simulink model "s_c_nbe_m1k"  (R2016b)
settings: Solver=VariableStepAuto  StartTime=0.0  StopTime=1000  RelTol=1e-3  EnableMultiTasking=on
undefined symbols (not defined in the file): Coeffs, fft_stages, n_taps, output_bits, pfb_coeff_gen_calc, xengbits
libraries: xbsIndex_r4 x23639, casper_library_misc x65, casper_library_scopes x4, xbsReplacements_r4 x4, xps_library x3
(part 34 of 198)

== system s_c_nbe_m1k/DDC/dec_fir_async1 ==
  sync_in : Inport
  dv_in : Inport  Port=2
  real1 : Inport  Port=3
  imag1 : Inport  Port=4
  real2 : Inport  Port=5
  imag2 : Inport  Port=6
  real3 : Inport  Port=7
  imag3 : Inport  Port=8
  real4 : Inport  Port=9
  imag4 : Inport  Port=10
  real5 : Inport  Port=11
  imag5 : Inport  Port=12
  real6 : Inport  Port=13
  imag6 : Inport  Port=14
  real7 : Inport  Port=15
  imag7 : Inport  Port=16
  real8 : Inport  Port=17
  imag8 : Inport  Port=18
  convert1 : xbsIndex_r4/Convert  gui_display_data_type=Fixed-point  arith_type="Signed  (2's comp)"  n_bits=10  bin_pt=9  float_type=Single  exp_bits=8  fraction_bits=24  quantization="Round  (unbiased: +/- Inf)"  overflow=Wrap  en=off  latency=7  pipeline=off  dbl_ovrd=off  block_type=convert
  convert2 : xbsIndex_r4/Convert  gui_display_data_type=Fixed-point  arith_type="Signed  (2's comp)"  n_bits=10  bin_pt=9  float_type=Single  exp_bits=8  fraction_bits=24  quantization="Round  (unbiased: +/- Inf)"  overflow=Wrap  en=off  latency=7  pipeline=off  dbl_ovrd=off  block_type=convert
  dv_delay : xbsIndex_r4/Delay  rst=off  infoeditControl=Selection of Reset will increase slice count due to use of real FFs and instead of SRLs  en=off  latency=70  reg_retiming=off  dbl_ovrd=off  block_type=delay
      settings: infoedit=Hardware notes: A delay line is a chain, each link of which is an SRL16 or SRL32 followed by a flip-flop.
  fir_col_async1 : Subsystem  AncestorBlock=casper_library_downconverter/fir_col_async  mask(fir_col_async){n_inputs=8, coeff=[-0.00042458 -0.00037722 -0.00032902 -0.00028149 -0.00023577 -0.00019291 -0.00015346   -0.000271], add_latency=7, mult_latency=7, coeff_bit_width=18, coeff_bin_pt=17, first_stage_hdl=on, adder_imp=DSP48, async=on, bus_input=off, input_width=0, input_bp=0, input_type=Signed, dbl=on}
      mask prompts: n_inputs "Inputs"; coeff "Coefficients"; add_latency "Add latency"; mult_latency "Mult Latency"; coeff_bit_width "Coefficient bit width"; coeff_bin_pt "Coefficient binary point"; first_stage_hdl "Implement first stage of adder trees on output as behavioural HDL"; adder_imp "Adder implementation"; async "Asynchronous ops"; bus_input "Bus input"; input_width "Input bitwidth"; input_bp "Input binary point"; input_type "Input datatype"; dbl "Double col"
      mask init:
      | fir_col_async_init(gcb);
      mask Help: eval('xlWeb(''http://casper.berkeley.edu/wiki/Fir_col'')')
      mask TypeOptions adder_imp: Behavioral | Fabric | DSP48
      mask Callback bus_input:
      | onoff = get_param(gcb, 'bus_input');
      | set_param_state(gcb, 'input_width', onoff)
      | set_param_state(gcb, 'input_bp', onoff)
      | set_param_state(gcb, 'input_type', onoff)
      mask TypeOptions input_type: Signed | Unsigned
  fir_col_async10 : Subsystem  AncestorBlock=casper_library_downconverter/fir_col_async  mask(fir_col_async){n_inputs=8, coeff=[0.0053089   0.0052932   0.0051518   0.0048953   0.0045363   0.0040891   0.0035695   0.0029938], add_latency=7, mult_latency=7, coeff_bit_width=18, coeff_bin_pt=17, first_stage_hdl=on, adder_imp=DSP48, async=on, bus_input=off, input_width=0, input_bp=0, input_type=Signed, dbl=on}
      mask prompts: n_inputs "Inputs"; coeff "Coefficients"; add_latency "Add latency"; mult_latency "Mult Latency"; coeff_bit_width "Coefficient bit width"; coeff_bin_pt "Coefficient binary point"; first_stage_hdl "Implement first stage of adder trees on output as behavioural HDL"; adder_imp "Adder implementation"; async "Asynchronous ops"; bus_input "Bus input"; input_width "Input bitwidth"; input_bp "Input binary point"; input_type "Input datatype"; dbl "Double col"
      mask init:
      | fir_col_async_init(gcb);
      mask Help: eval('xlWeb(''http://casper.berkeley.edu/wiki/Fir_col'')')
      mask TypeOptions adder_imp: Behavioral | Fabric | DSP48
      mask Callback bus_input:
      | onoff = get_param(gcb, 'bus_input');
      | set_param_state(gcb, 'input_width', onoff)
      | set_param_state(gcb, 'input_bp', onoff)
      | set_param_state(gcb, 'input_type', onoff)
      mask TypeOptions input_type: Signed | Unsigned
  fir_col_async11 : Subsystem  AncestorBlock=casper_library_downconverter/fir_col_async  mask(fir_col_async){n_inputs=8, coeff=[0.00060481   0.0016168   0.0025297    0.003328   0.0039999   0.0045369   0.0049344   0.0051911], add_latency=7, mult_latency=7, coeff_bit_width=18, coeff_bin_pt=17, first_stage_hdl=on, adder_imp=DSP48, async=on, bus_input=off, input_width=0, input_bp=0, input_type=Signed, dbl=on}
      mask prompts: n_inputs "Inputs"; coeff "Coefficients"; add_latency "Add latency"; mult_latency "Mult Latency"; coeff_bit_width "Coefficient bit width"; coeff_bin_pt "Coefficient binary point"; first_stage_hdl "Implement first stage of adder trees on output as behavioural HDL"; adder_imp "Adder implementation"; async "Asynchronous ops"; bus_input "Bus input"; input_width "Input bitwidth"; input_bp "Input binary point"; input_type "Input datatype"; dbl "Double col"
      mask init:
      | fir_col_async_init(gcb);
      mask Help: eval('xlWeb(''http://casper.berkeley.edu/wiki/Fir_col'')')
      mask TypeOptions adder_imp: Behavioral | Fabric | DSP48
      mask Callback bus_input:
      | onoff = get_param(gcb, 'bus_input');
      | set_param_state(gcb, 'input_width', onoff)
      | set_param_state(gcb, 'input_bp', onoff)
      | set_param_state(gcb, 'input_type', onoff)
      mask TypeOptions input_type: Signed | Unsigned
  fir_col_async12 : Subsystem  AncestorBlock=casper_library_downconverter/fir_col_async  mask(fir_col_async){n_inputs=8, coeff=[-0.0082442  -0.0073287  -0.0062974  -0.0051819  -0.0040135  -0.0028225  -0.0016382 -0.00048749], add_latency=7, mult_latency=7, coeff_bit_width=18, coeff_bin_pt=17, first_stage_hdl=on, adder_imp=DSP48, async=on, bus_input=off, input_width=0, input_bp=0, input_type=Signed, dbl=on}
      mask prompts: n_inputs "Inputs"; coeff "Coefficients"; add_latency "Add latency"; mult_latency "Mult Latency"; coeff_bit_width "Coefficient bit width"; coeff_bin_pt "Coefficient binary point"; first_stage_hdl "Implement first stage of adder trees on output as behavioural HDL"; adder_imp "Adder implementation"; async "Asynchronous ops"; bus_input "Bus input"; input_width "Input bitwidth"; input_bp "Input binary point"; input_type "Input datatype"; dbl "Double col"
      mask init:
      | fir_col_async_init(gcb);
      mask Help: eval('xlWeb(''http://casper.berkeley.edu/wiki/Fir_col'')')
      mask TypeOptions adder_imp: Behavioral | Fabric | DSP48
      mask Callback bus_input:
      | onoff = get_param(gcb, 'bus_input');
      | set_param_state(gcb, 'input_width', onoff)
      | set_param_state(gcb, 'input_bp', onoff)
      | set_param_state(gcb, 'input_type', onoff)
      mask TypeOptions input_type: Signed | Unsigned
  fir_col_async13 : Subsystem  AncestorBlock=casper_library_downconverter/fir_col_async  mask(fir_col_async){n_inputs=8, coeff=[-0.0080689  -0.0090238   -0.009681   -0.010051   -0.010148  -0.0099918  -0.0096048  -0.0090129], add_latency=7, mult_latency=7, coeff_bit_width=18, coeff_bin_pt=17, first_stage_hdl=on, adder_imp=DSP48, async=on, bus_input=off, input_width=0, input_bp=0, input_type=Signed, dbl=on}
      mask prompts: n_inputs "Inputs"; coeff "Coefficients"; add_latency "Add latency"; mult_latency "Mult Latency"; coeff_bit_width "Coefficient bit width"; coeff_bin_pt "Coefficient binary point"; first_stage_hdl "Implement first stage of adder trees on output as behavioural HDL"; adder_imp "Adder implementation"; async "Asynchronous ops"; bus_input "Bus input"; input_width "Input bitwidth"; input_bp "Input binary point"; input_type "Input datatype"; dbl "Double col"
      mask init:
      | fir_col_async_init(gcb);
      mask Help: eval('xlWeb(''http://casper.berkeley.edu/wiki/Fir_col'')')
      mask TypeOptions adder_imp: Behavioral | Fabric | DSP48
      mask Callback bus_input:
      | onoff = get_param(gcb, 'bus_input');
      | set_param_state(gcb, 'input_width', onoff)
      | set_param_state(gcb, 'input_bp', onoff)
      | set_param_state(gcb, 'input_type', onoff)
      mask TypeOptions input_type: Signed | Unsigned
  fir_col_async14 : Subsystem  AncestorBlock=casper_library_downconverter/fir_col_async  mask(fir_col_async){n_inputs=8, coeff=[0.0097893   0.0067161    0.003832   0.0011688  -0.0012463  -0.0033914  -0.0052499  -0.0068109], add_latency=7, mult_latency=7, coeff_bit_width=18, coeff_bin_pt=17, first_stage_hdl=on, adder_imp=DSP48, async=on, bus_input=off, input_width=0, input_bp=0, input_type=Signed, dbl=on}
      mask prompts: n_inputs "Inputs"; coeff "Coefficients"; add_latency "Add latency"; mult_latency "Mult Latency"; coeff_bit_width "Coefficient bit width"; coeff_bin_pt "Coefficient binary point"; first_stage_hdl "Implement first stage of adder trees on output as behavioural HDL"; adder_imp "Adder implementation"; async "Asynchronous ops"; bus_input "Bus input"; input_width "Input bitwidth"; input_bp "Input binary point"; input_type "Input datatype"; dbl "Double col"
      mask init:
      | fir_col_async_init(gcb);
      mask Help: eval('xlWeb(''http://casper.berkeley.edu/wiki/Fir_col'')')
      mask TypeOptions adder_imp: Behavioral | Fabric | DSP48
      mask Callback bus_input:
      | onoff = get_param(gcb, 'bus_input');
      | set_param_state(gcb, 'input_width', onoff)
      | set_param_state(gcb, 'input_bp', onoff)
      | set_param_state(gcb, 'input_type', onoff)
      mask TypeOptions input_type: Signed | Unsigned
  fir_col_async15 : Subsystem  AncestorBlock=casper_library_downconverter/fir_col_async  mask(fir_col_async){n_inputs=8, coeff=[0.03623    0.033172    0.029949    0.026609    0.023197    0.019764    0.016355    0.013015], add_latency=7, mult_latency=7, coeff_bit_width=18, coeff_bin_pt=17, first_stage_hdl=on, adder_imp=DSP48, async=on, bus_input=off, input_width=0, input_bp=0, input_type=Signed, dbl=on}
      mask prompts: n_inputs "Inputs"; coeff "Coefficients"; add_latency "Add latency"; mult_latency "Mult Latency"; coeff_bit_width "Coefficient bit width"; coeff_bin_pt "Coefficient binary point"; first_stage_hdl "Implement first stage of adder trees on output as behavioural HDL"; adder_imp "Adder implementation"; async "Asynchronous ops"; bus_input "Bus input"; input_width "Input bitwidth"; input_bp "Input binary point"; input_type "Input datatype"; dbl "Double col"
      mask init:
      | fir_col_async_init(gcb);
      mask Help: eval('xlWeb(''http://casper.berkeley.edu/wiki/Fir_col'')')
      mask TypeOptions adder_imp: Behavioral | Fabric | DSP48
      mask Callback bus_input:
      | onoff = get_param(gcb, 'bus_input');
      | set_param_state(gcb, 'input_width', onoff)
      | set_param_state(gcb, 'input_bp', onoff)
      | set_param_state(gcb, 'input_type', onoff)
      mask TypeOptions input_type: Signed | Unsigned
  fir_col_async16 : Subsystem  AncestorBlock=casper_library_downconverter/fir_col_async  mask(fir_col_async){n_inputs=8, coeff=[0.050061     0.04964    0.048805    0.047569     0.04595    0.043974    0.041672    0.039077], add_latency=7, mult_latency=7, coeff_bit_width=18, coeff_bin_pt=17, first_stage_hdl=on, adder_imp=DSP48, async=on, bus_input=off, input_width=0, input_bp=0, input_type=Signed, dbl=on}
      mask prompts: n_inputs "Inputs"; coeff "Coefficients"; add_latency "Add latency"; mult_latency "Mult Latency"; coeff_bit_width "Coefficient bit width"; coeff_bin_pt "Coefficient binary point"; first_stage_hdl "Implement first stage of adder trees on output as behavioural HDL"; adder_imp "Adder implementation"; async "Asynchronous ops"; bus_input "Bus input"; input_width "Input bitwidth"; input_bp "Input binary point"; input_type "Input datatype"; dbl "Double col"
      mask init:
      | fir_col_async_init(gcb);
      mask Help: eval('xlWeb(''http://casper.berkeley.edu/wiki/Fir_col'')')
      mask TypeOptions adder_imp: Behavioral | Fabric | DSP48
      mask Callback bus_input:
      | onoff = get_param(gcb, 'bus_input');
      | set_param_state(gcb, 'input_width', onoff)
      | set_param_state(gcb, 'input_bp', onoff)
      | set_param_state(gcb, 'input_type', onoff)
      mask TypeOptions input_type: Signed | Unsigned
  fir_col_async2 : Subsystem  AncestorBlock=casper_library_downconverter/fir_col_async  mask(fir_col_async){n_inputs=8, coeff=[-0.00057574 -0.00059619   -0.000602 -0.00059433 -0.00057544  -0.0005472 -0.00051125 -0.00046978], add_latency=7, mult_latency=7, coeff_bit_width=18, coeff_bin_pt=17, first_stage_hdl=on, adder_imp=DSP48, async=on, bus_input=off, input_width=0, input_bp=0, input_type=Signed, dbl=on}
      mask prompts: n_inputs "Inputs"; coeff "Coefficients"; add_latency "Add latency"; mult_latency "Mult Latency"; coeff_bit_width "Coefficient bit width"; coeff_bin_pt "Coefficient binary point"; first_stage_hdl "Implement first stage of adder trees on output as behavioural HDL"; adder_imp "Adder implementation"; async "Asynchronous ops"; bus_input "Bus input"; input_width "Input bitwidth"; input_bp "Input binary point"; input_type "Input datatype"; dbl "Double col"
      mask init:
      | fir_col_async_init(gcb);
      mask Help: eval('xlWeb(''http://casper.berkeley.edu/wiki/Fir_col'')')
      mask TypeOptions adder_imp: Behavioral | Fabric | DSP48
      mask Callback bus_input:
      | onoff = get_param(gcb, 'bus_input');
      | set_param_state(gcb, 'input_width', onoff)
      | set_param_state(gcb, 'input_bp', onoff)
      | set_param_state(gcb, 'input_type', onoff)
      mask TypeOptions input_type: Signed | Unsigned
  fir_col_async3 : Subsystem  AncestorBlock=casper_library_downconverter/fir_col_async  mask(fir_col_async){n_inputs=8, coeff=[0.00024451  7.6958e-05 -7.3315e-05 -0.00020513 -0.00031757 -0.00041046 -0.00048394 -0.00053871], add_latency=7, mult_latency=7, coeff_bit_width=18, coeff_bin_pt=17, first_stage_hdl=on, adder_imp=DSP48, async=on, bus_input=off, input_width=0, input_bp=0, input_type=Signed, dbl=on}
      mask prompts: n_inputs "Inputs"; coeff "Coefficients"; add_latency "Add latency"; mult_latency "Mult Latency"; coeff_bit_width "Coefficient bit width"; coeff_bin_pt "Coefficient binary point"; first_stage_hdl "Implement first stage of adder trees on output as behavioural HDL"; adder_imp "Adder implementation"; async "Asynchronous ops"; bus_input "Bus input"; input_width "Input bitwidth"; input_bp "Input binary point"; input_type "Input datatype"; dbl "Double col"
      mask init:
      | fir_col_async_init(gcb);
      mask Help: eval('xlWeb(''http://casper.berkeley.edu/wiki/Fir_col'')')
      mask TypeOptions adder_imp: Behavioral | Fabric | DSP48
      mask Callback bus_input:
      | onoff = get_param(gcb, 'bus_input');
      | set_param_state(gcb, 'input_width', onoff)
      | set_param_state(gcb, 'input_bp', onoff)
      | set_param_state(gcb, 'input_type', onoff)
      mask TypeOptions input_type: Signed | Unsigned
  fir_col_async4 : Subsystem  AncestorBlock=casper_library_downconverter/fir_col_async  mask(fir_col_async){n_inputs=8, coeff=[0.0018729    0.001677     0.00147   0.0012565   0.0010415  0.00082907  0.00062325   0.0004274], add_latency=7, mult_latency=7, coeff_bit_width=18, coeff_bin_pt=17, first_stage_hdl=on, adder_imp=DSP48, async=on, bus_input=off, input_width=0, input_bp=0, input_type=Signed, dbl=on}
      mask prompts: n_inputs "Inputs"; coeff "Coefficients"; add_latency "Add latency"; mult_latency "Mult Latency"; coeff_bit_width "Coefficient bit width"; coeff_bin_pt "Coefficient binary point"; first_stage_hdl "Implement first stage of adder trees on output as behavioural HDL"; adder_imp "Adder implementation"; async "Asynchronous ops"; bus_input "Bus input"; input_width "Input bitwidth"; input_bp "Input binary point"; input_type "Input datatype"; dbl "Double col"
      mask init:
      | fir_col_async_init(gcb);
      mask Help: eval('xlWeb(''http://casper.berkeley.edu/wiki/Fir_col'')')
      mask TypeOptions adder_imp: Behavioral | Fabric | DSP48
      mask Callback bus_input:
      | onoff = get_param(gcb, 'bus_input');
      | set_param_state(gcb, 'input_width', onoff)
      | set_param_state(gcb, 'input_bp', onoff)
      | set_param_state(gcb, 'input_type', onoff)
      mask TypeOptions input_type: Signed | Unsigned
  fir_col_async5 : Subsystem  AncestorBlock=casper_library_downconverter/fir_col_async  mask(fir_col_async){n_inputs=8, coeff=[0.002468   0.0025259   0.0025398   0.0025118   0.0024451   0.0023435   0.0022111   0.0020526], add_latency=7, mult_latency=7, coeff_bit_width=18, coeff_bin_pt=17, first_stage_hdl=on, adder_imp=DSP48, async=on, bus_input=off, input_width=0, input_bp=0, input_type=Signed, dbl=on}
      mask prompts: n_inputs "Inputs"; coeff "Coefficients"; add_latency "Add latency"; mult_latency "Mult Latency"; coeff_bit_width "Coefficient bit width"; coeff_bin_pt "Coefficient binary point"; first_stage_hdl "Implement first stage of adder trees on output as behavioural HDL"; adder_imp "Adder implementation"; async "Asynchronous ops"; bus_input "Bus input"; input_width "Input bitwidth"; input_bp "Input binary point"; input_type "Input datatype"; dbl "Double col"
      mask init:
      | fir_col_async_init(gcb);
      mask Help: eval('xlWeb(''http://casper.berkeley.edu/wiki/Fir_col'')')
      mask TypeOptions adder_imp: Behavioral | Fabric | DSP48
      mask Callback bus_input:
      | onoff = get_param(gcb, 'bus_input');
      | set_param_state(gcb, 'input_width', onoff)
      | set_param_state(gcb, 'input_bp', onoff)
      | set_param_state(gcb, 'input_type', onoff)
      mask TypeOptions input_type: Signed | Unsigned
  fir_col_async6 : Subsystem  AncestorBlock=casper_library_downconverter/fir_col_async  mask(fir_col_async){n_inputs=8, coeff=[0.00046831  0.00084053   0.0011876   0.0015031   0.0017821   0.0020204   0.0022151   0.0023645], add_latency=7, mult_latency=7, coeff_bit_width=18, coeff_bin_pt=17, first_stage_hdl=on, adder_imp=DSP48, async=on, bus_input=off, input_width=0, input_bp=0, input_type=Signed, dbl=on}
      mask prompts: n_inputs "Inputs"; coeff "Coefficients"; add_latency "Add latency"; mult_latency "Mult Latency"; coeff_bit_width "Coefficient bit width"; coeff_bin_pt "Coefficient binary point"; first_stage_hdl "Implement first stage of adder trees on output as behavioural HDL"; adder_imp "Adder implementation"; async "Asynchronous ops"; bus_input "Bus input"; input_width "Input bitwidth"; input_bp "Input binary point"; input_type "Input datatype"; dbl "Double col"
      mask init:
      | fir_col_async_init(gcb);
      mask Help: eval('xlWeb(''http://casper.berkeley.edu/wiki/Fir_col'')')
      mask TypeOptions adder_imp: Behavioral | Fabric | DSP48
      mask Callback bus_input:
      | onoff = get_param(gcb, 'bus_input');
      | set_param_state(gcb, 'input_width', onoff)
      | set_param_state(gcb, 'input_bp', onoff)
      | set_param_state(gcb, 'input_type', onoff)
      mask TypeOptions input_type: Signed | Unsigned
  fir_col_async7 : Subsystem  AncestorBlock=casper_library_downconverter/fir_col_async  mask(fir_col_async){n_inputs=8, coeff=[-0.0024155   -0.002151  -0.0018401  -0.0014922  -0.0011167 -0.00072347  -0.0003221   7.805e-05], add_latency=7, mult_latency=7, coeff_bit_width=18, coeff_bin_pt=17, first_stage_hdl=on, adder_imp=DSP48, async=on, bus_input=off, input_width=0, input_bp=0, input_type=Signed, dbl=on}
      mask prompts: n_inputs "Inputs"; coeff "Coefficients"; add_latency "Add latency"; mult_latency "Mult Latency"; coeff_bit_width "Coefficient bit width"; coeff_bin_pt "Coefficient binary point"; first_stage_hdl "Implement first stage of adder trees on output as behavioural HDL"; adder_imp "Adder implementation"; async "Asynchronous ops"; bus_input "Bus input"; input_width "Input bitwidth"; input_bp "Input binary point"; input_type "Input datatype"; dbl "Double col"
      mask init:
      | fir_col_async_init(gcb);
      mask Help: eval('xlWeb(''http://casper.berkeley.edu/wiki/Fir_col'')')
      mask TypeOptions adder_imp: Behavioral | Fabric | DSP48
      mask Callback bus_input:
      | onoff = get_param(gcb, 'bus_input');
      | set_param_state(gcb, 'input_width', onoff)
      | set_param_state(gcb, 'input_bp', onoff)
      | set_param_state(gcb, 'input_type', onoff)
      mask TypeOptions input_type: Signed | Unsigned
  fir_col_async8 : Subsystem  AncestorBlock=casper_library_downconverter/fir_col_async  mask(fir_col_async){n_inputs=8, coeff=[-0.0020709  -0.0023853  -0.0026213  -0.0027769  -0.0028523  -0.0028494  -0.0027719   -0.002625], add_latency=7, mult_latency=7, coeff_bit_width=18, coeff_bin_pt=17, first_stage_hdl=on, adder_imp=DSP48, async=on, bus_input=off, input_width=0, input_bp=0, input_type=Signed, dbl=on}
      mask prompts: n_inputs "Inputs"; coeff "Coefficients"; add_latency "Add latency"; mult_latency "Mult Latency"; coeff_bit_width "Coefficient bit width"; coeff_bin_pt "Coefficient binary point"; first_stage_hdl "Implement first stage of adder trees on output as behavioural HDL"; adder_imp "Adder implementation"; async "Asynchronous ops"; bus_input "Bus input"; input_width "Input bitwidth"; input_bp "Input binary point"; input_type "Input datatype"; dbl "Double col"
      mask init:
      | fir_col_async_init(gcb);
      mask Help: eval('xlWeb(''http://casper.berkeley.edu/wiki/Fir_col'')')
      mask TypeOptions adder_imp: Behavioral | Fabric | DSP48
      mask Callback bus_input:
      | onoff = get_param(gcb, 'bus_input');
      | set_param_state(gcb, 'input_width', onoff)
      | set_param_state(gcb, 'input_bp', onoff)
      | set_param_state(gcb, 'input_type', onoff)
      mask TypeOptions input_type: Signed | Unsigned
  fir_col_async9 : Subsystem  AncestorBlock=casper_library_downconverter/fir_col_async  mask(fir_col_async){n_inputs=8, coeff=[0.002379   0.0017422   0.0010999    0.000468 -0.00013873 -0.00070691  -0.0012246   -0.001682], add_latency=7, mult_latency=7, coeff_bit_width=18, coeff_bin_pt=17, first_stage_hdl=on, adder_imp=DSP48, async=on, bus_input=off, input_width=0, input_bp=0, input_type=Signed, dbl=on}
      mask prompts: n_inputs "Inputs"; coeff "Coefficients"; add_latency "Add latency"; mult_latency "Mult Latency"; coeff_bit_width "Coefficient bit width"; coeff_bin_pt "Coefficient binary point"; first_stage_hdl "Implement first stage of adder trees on output as behavioural HDL"; adder_imp "Adder implementation"; async "Asynchronous ops"; bus_input "Bus input"; input_width "Input bitwidth"; input_bp "Input binary point"; input_type "Input datatype"; dbl "Double col"
      mask init:
      | fir_col_async_init(gcb);
      mask Help: eval('xlWeb(''http://casper.berkeley.edu/wiki/Fir_col'')')
      mask TypeOptions adder_imp: Behavioral | Fabric | DSP48
      mask Callback bus_input:
      | onoff = get_param(gcb, 'bus_input');
      | set_param_state(gcb, 'input_width', onoff)
      | set_param_state(gcb, 'input_bp', onoff)
      | set_param_state(gcb, 'input_type', onoff)
      mask TypeOptions input_type: Signed | Unsigned
  imag_sum : Subsystem  AncestorBlock=casper_library_misc/adder_tree  mask(adder_tree){n_inputs=16, latency=7, adder_imp=DSP48, first_stage_hdl=off, floating_point=off, float_type=single, frac_width=0, exp_width=0}
      mask prompts: n_inputs "Number of Inputs"; latency "Add Latency"; adder_imp "Adder implementation"; first_stage_hdl "Use behavioural HDL for first stage of adders"; floating_point "floating point"; float_type "float type"; frac_width "fraction length"; exp_width "exponent length"
      mask help:
      | Sums all inputs using a tree of adds and delays.
      |
      | Number of inputs: The number of inputs to the block to be summed
      | Add latency: The number of clock cycles to perform one addition (affects timing)..
      | Adder implementation: choice of fabric or DSP48E core, or behavioral HDL
      | Use behavioural HDL for first stage of adders: Causes the first stage of adders to be absorbed into DSP blocks if multipliers precede them (Virtex 5). Overrides Adder implementation
      mask init:
      | adder_tree_init(gcb, ...
      |     'n_inputs', n_inputs, ...
      |     'latency', latency, ...
      |     'adder_imp', adder_imp, ...
      |     'floating_point', floating_point, ...
      |     'float_type', float_type, ...
      |     'exp_width', exp_width, ...
      |     'frac_width', frac_width, ...     
      |     'first_stage_hdl', first_stage_hdl);
      settings: AttributesFormatString=latency 28
      mask Help: eval('xlWeb(''http://casper.berkeley.edu/wiki/Adder_tree'')')
      mask TypeOptions adder_imp: Behavioral | Fabric | DSP48
      mask Callback floating_point:
      | onoff = get_param(gcb, 'floating_point');
      | if strcmp(onoff,'on')
      |     enable_fixpt = 'off'
      |     set_param_state(gcb, 'float_type', 'on')
      | 
      |     f_type = get_param(gcb, 'float_type')
      |     if strcmp(f_type,'custom')
      |         set_param_state(gcb, 'exp_width', 'on')
      |         set_param_state(gcb, 'frac_width', 'on')
      |     else
      |         set_param_state(gcb, 'exp_width', 'off')
      |         set_param_state(gcb, 'frac_width', 'off')
      |     end
      | 
      | 
      | else
      |     enable_fixpt = 'on'
      |     set_param_state(gcb, 'float_type', 'off')
      |     set_param_state(gcb, 'exp_width', 'off')
      |     set_param_state(gcb, 'frac_width', 'off')
      | end
      mask TypeOptions float_type: single | custom
      mask Callback float_type:
      | f_type = get_param(gcb, 'float_type')
      | if strcmp(f_type,'custom')
      |     set_param_state(gcb, 'exp_width', 'on')
      |     set_param_state(gcb, 'frac_width', 'on')
      | else
      |     set_param_state(gcb, 'exp_width', 'off')
      |     set_param_state(gcb, 'frac_width', 'off')
      | end
  real_sum : Subsystem  AncestorBlock=casper_library_misc/adder_tree  mask(adder_tree){n_inputs=16, latency=7, adder_imp=DSP48, first_stage_hdl=off, floating_point=off, float_type=single, frac_width=0, exp_width=0}
      mask prompts: n_inputs "Number of Inputs"; latency "Add Latency"; adder_imp "Adder implementation"; first_stage_hdl "Use behavioural HDL for first stage of adders"; floating_point "floating point"; float_type "float type"; frac_width "fraction length"; exp_width "exponent length"
      mask help:
      | Sums all inputs using a tree of adds and delays.
      |
      | Number of inputs: The number of inputs to the block to be summed
      | Add latency: The number of clock cycles to perform one addition (affects timing)..
      | Adder implementation: choice of fabric or DSP48E core, or behavioral HDL
      | Use behavioural HDL for first stage of adders: Causes the first stage of adders to be absorbed into DSP blocks if multipliers precede them (Virtex 5). Overrides Adder implementation
      mask init: same as s_c_nbe_m1k/DDC/dec_fir_async1/imag_sum
      settings: AttributesFormatString=latency 28
      mask Help: eval('xlWeb(''http://casper.berkeley.edu/wiki/Adder_tree'')')
      mask TypeOptions adder_imp: Behavioral | Fabric | DSP48
      mask Callback floating_point:
      | onoff = get_param(gcb, 'floating_point');
      | if strcmp(onoff,'on')
      |     enable_fixpt = 'off'
      |     set_param_state(gcb, 'float_type', 'on')
      | 
      |     f_type = get_param(gcb, 'float_type')
      |     if strcmp(f_type,'custom')
      |         set_param_state(gcb, 'exp_width', 'on')
      |         set_param_state(gcb, 'frac_width', 'on')
      |     else
      |         set_param_state(gcb, 'exp_width', 'off')
      |         set_param_state(gcb, 'frac_width', 'off')
      |     end
      | 
      | 
      | else
      |     enable_fixpt = 'on'
      |     set_param_state(gcb, 'float_type', 'off')
      |     set_param_state(gcb, 'exp_width', 'off')
      |     set_param_state(gcb, 'frac_width', 'off')
      | end
      mask TypeOptions float_type: single | custom
      mask Callback float_type:
      | f_type = get_param(gcb, 'float_type')
      | if strcmp(f_type,'custom')
      |     set_param_state(gcb, 'exp_width', 'on')
      |     set_param_state(gcb, 'frac_width', 'on')
      | else
      |     set_param_state(gcb, 'exp_width', 'off')
      |     set_param_state(gcb, 'frac_width', 'off')
      | end
  ri_to_c : casper_library_misc/ri_to_c
  shift1 : xbsIndex_r4/Shift  shift_dir=Left  shift_bits=1  en=off  latency=1  precision=Full  arith_type="Signed  (2's comp)"  n_bits=16  bin_pt=14  quantization=Truncate  overflow=Wrap  dbl_ovrd=off  block_type=shift
  shift2 : xbsIndex_r4/Shift  shift_dir=Left  shift_bits=1  en=off  latency=1  precision=Full  arith_type="Signed  (2's comp)"  n_bits=16  bin_pt=14  quantization=Truncate  overflow=Wrap  dbl_ovrd=off  block_type=shift
  sync_delay : xbsIndex_r4/Delay  rst=off  infoeditControl=Selection of Reset will increase slice count due to use of real FFs and instead of SRLs  en=off  latency=42  reg_retiming=off  dbl_ovrd=off  block_type=delay
      settings: infoedit=Hardware notes: A delay line is a chain, each link of which is an SRL16 or SRL32 followed by a flip-flop.
  sync_out : Outport
  dout : Outport  Port=2
  dv_out : Outport  Port=3
  wires:
  sync_in/1 -> sync_delay/1
  dv_in/1 -> dv_delay/1, fir_col_async1/33(dv), fir_col_async2/33(dv), fir_col_async3/33(dv), fir_col_async4/33(dv), fir_col_async5/33(dv), fir_col_async6/33(dv), fir_col_async7/33(dv), fir_col_async8/33(dv), fir_col_async9/33(dv), fir_col_async10/33(dv), fir_col_async11/33(dv), fir_col_async12/33(dv), fir_col_async13/33(dv), fir_col_async14/33(dv), fir_col_async15/33(dv), fir_col_async16/33(dv)
  dv_delay/1 -> dv_out/1
  real1/1 -> fir_col_async1/1(real1)
  imag1/1 -> fir_col_async1/2(imag1)
  real2/1 -> fir_col_async1/3(real2)
  imag2/1 -> fir_col_async1/4(imag2)
  real3/1 -> fir_col_async1/5(real3)
  imag3/1 -> fir_col_async1/6(imag3)
  real4/1 -> fir_col_async1/7(real4)
  imag4/1 -> fir_col_async1/8(imag4)
  real5/1 -> fir_col_async1/9(real5)
  imag5/1 -> fir_col_async1/10(imag5)
  real6/1 -> fir_col_async1/11(real6)
  imag6/1 -> fir_col_async1/12(imag6)
  real7/1 -> fir_col_async1/13(real7)
  imag7/1 -> fir_col_async1/14(imag7)
  real8/1 -> fir_col_async1/15(real8)
  imag8/1 -> fir_col_async1/16(imag8)
  fir_col_async1/33(real_sum) -> real_sum/2(din1)
  fir_col_async1/34(imag_sum) -> imag_sum/2(din1)
  fir_col_async1/1(real_out1) -> fir_col_async2/1(real1)
  fir_col_async1/2(imag_out1) -> fir_col_async2/2(imag1)
  fir_col_async1/3(real_out2) -> fir_col_async2/3(real2)
  fir_col_async1/4(imag_out2) -> fir_col_async2/4(imag2)
  fir_col_async1/5(real_out3) -> fir_col_async2/5(real3)
  fir_col_async1/6(imag_out3) -> fir_col_async2/6(imag3)
  fir_col_async1/7(real_out4) -> fir_col_async2/7(real4)
  fir_col_async1/8(imag_out4) -> fir_col_async2/8(imag4)
  fir_col_async1/9(real_out5) -> fir_col_async2/9(real5)
  fir_col_async1/10(imag_out5) -> fir_col_async2/10(imag5)
  fir_col_async1/11(real_out6) -> fir_col_async2/11(real6)
  fir_col_async1/12(imag_out6) -> fir_col_async2/12(imag6)
  fir_col_async1/13(real_out7) -> fir_col_async2/13(real7)
  fir_col_async1/14(imag_out7) -> fir_col_async2/14(imag7)
  fir_col_async1/15(real_out8) -> fir_col_async2/15(real8)
  fir_col_async1/16(imag_out8) -> fir_col_async2/16(imag8)
  fir_col_async2/33(real_sum) -> real_sum/3(din2)
  fir_col_async2/34(imag_sum) -> imag_sum/3(din2)
  fir_col_async2/1(real_out1) -> fir_col_async3/1(real1)
  fir_col_async2/2(imag_out1) -> fir_col_async3/2(imag1)
  fir_col_async2/3(real_out2) -> fir_col_async3/3(real2)
  fir_col_async2/4(imag_out2) -> fir_col_async3/4(imag2)
  fir_col_async2/5(real_out3) -> fir_col_async3/5(real3)
  fir_col_async2/6(imag_out3) -> fir_col_async3/6(imag3)
  fir_col_async2/7(real_out4) -> fir_col_async3/7(real4)
  fir_col_async2/8(imag_out4) -> fir_col_async3/8(imag4)
  fir_col_async2/9(real_out5) -> fir_col_async3/9(real5)
  fir_col_async2/10(imag_out5) -> fir_col_async3/10(imag5)
  fir_col_async2/11(real_out6) -> fir_col_async3/11(real6)
  fir_col_async2/12(imag_out6) -> fir_col_async3/12(imag6)
  fir_col_async2/13(real_out7) -> fir_col_async3/13(real7)
  fir_col_async2/14(imag_out7) -> fir_col_async3/14(imag7)
  fir_col_async2/15(real_out8) -> fir_col_async3/15(real8)
  fir_col_async2/16(imag_out8) -> fir_col_async3/16(imag8)
  fir_col_async3/33(real_sum) -> real_sum/4(din3)
  fir_col_async3/34(imag_sum) -> imag_sum/4(din3)
  fir_col_async3/1(real_out1) -> fir_col_async4/1(real1)
  fir_col_async3/2(imag_out1) -> fir_col_async4/2(imag1)
  fir_col_async3/3(real_out2) -> fir_col_async4/3(real2)
  fir_col_async3/4(imag_out2) -> fir_col_async4/4(imag2)
  fir_col_async3/5(real_out3) -> fir_col_async4/5(real3)
  fir_col_async3/6(imag_out3) -> fir_col_async4/6(imag3)
  fir_col_async3/7(real_out4) -> fir_col_async4/7(real4)
  fir_col_async3/8(imag_out4) -> fir_col_async4/8(imag4)
  fir_col_async3/9(real_out5) -> fir_col_async4/9(real5)
  fir_col_async3/10(imag_out5) -> fir_col_async4/10(imag5)
  fir_col_async3/11(real_out6) -> fir_col_async4/11(real6)
  fir_col_async3/12(imag_out6) -> fir_col_async4/12(imag6)
  fir_col_async3/13(real_out7) -> fir_col_async4/13(real7)
  fir_col_async3/14(imag_out7) -> fir_col_async4/14(imag7)
  fir_col_async3/15(real_out8) -> fir_col_async4/15(real8)
  fir_col_async3/16(imag_out8) -> fir_col_async4/16(imag8)
  fir_col_async4/33(real_sum) -> real_sum/5(din4)
  fir_col_async4/34(imag_sum) -> imag_sum/5(din4)
  fir_col_async4/1(real_out1) -> fir_col_async5/1(real1)
  fir_col_async4/2(imag_out1) -> fir_col_async5/2(imag1)
  fir_col_async4/3(real_out2) -> fir_col_async5/3(real2)
  fir_col_async4/4(imag_out2) -> fir_col_async5/4(imag2)
  fir_col_async4/5(real_out3) -> fir_col_async5/5(real3)
  fir_col_async4/6(imag_out3) -> fir_col_async5/6(imag3)
  fir_col_async4/7(real_out4) -> fir_col_async5/7(real4)
  fir_col_async4/8(imag_out4) -> fir_col_async5/8(imag4)
  fir_col_async4/9(real_out5) -> fir_col_async5/9(real5)
  fir_col_async4/10(imag_out5) -> fir_col_async5/10(imag5)
  fir_col_async4/11(real_out6) -> fir_col_async5/11(real6)
  fir_col_async4/12(imag_out6) -> fir_col_async5/12(imag6)
  fir_col_async4/13(real_out7) -> fir_col_async5/13(real7)
  fir_col_async4/14(imag_out7) -> fir_col_async5/14(imag7)
  fir_col_async4/15(real_out8) -> fir_col_async5/15(real8)
  fir_col_async4/16(imag_out8) -> fir_col_async5/16(imag8)
  fir_col_async5/33(real_sum) -> real_sum/6(din5)
  fir_col_async5/34(imag_sum) -> imag_sum/6(din5)
  fir_col_async5/1(real_out1) -> fir_col_async6/1(real1)
  fir_col_async5/2(imag_out1) -> fir_col_async6/2(imag1)
  fir_col_async5/3(real_out2) -> fir_col_async6/3(real2)
  fir_col_async5/4(imag_out2) -> fir_col_async6/4(imag2)
  fir_col_async5/5(real_out3) -> fir_col_async6/5(real3)
  fir_col_async5/6(imag_out3) -> fir_col_async6/6(imag3)
  fir_col_async5/7(real_out4) -> fir_col_async6/7(real4)
  fir_col_async5/8(imag_out4) -> fir_col_async6/8(imag4)
  fir_col_async5/9(real_out5) -> fir_col_async6/9(real5)
  fir_col_async5/10(imag_out5) -> fir_col_async6/10(imag5)
  fir_col_async5/11(real_out6) -> fir_col_async6/11(real6)
  fir_col_async5/12(imag_out6) -> fir_col_async6/12(imag6)
  fir_col_async5/13(real_out7) -> fir_col_async6/13(real7)
  fir_col_async5/14(imag_out7) -> fir_col_async6/14(imag7)
  fir_col_async5/15(real_out8) -> fir_col_async6/15(real8)
  fir_col_async5/16(imag_out8) -> fir_col_async6/16(imag8)
  fir_col_async6/33(real_sum) -> real_sum/7(din6)
  fir_col_async6/34(imag_sum) -> imag_sum/7(din6)
  fir_col_async6/1(real_out1) -> fir_col_async7/1(real1)
  fir_col_async6/2(imag_out1) -> fir_col_async7/2(imag1)
  fir_col_async6/3(real_out2) -> fir_col_async7/3(real2)
  fir_col_async6/4(imag_out2) -> fir_col_async7/4(imag2)
  fir_col_async6/5(real_out3) -> fir_col_async7/5(real3)
  fir_col_async6/6(imag_out3) -> fir_col_async7/6(imag3)
  fir_col_async6/7(real_out4) -> fir_col_async7/7(real4)
  fir_col_async6/8(imag_out4) -> fir_col_async7/8(imag4)
  fir_col_async6/9(real_out5) -> fir_col_async7/9(real5)
  fir_col_async6/10(imag_out5) -> fir_col_async7/10(imag5)
  fir_col_async6/11(real_out6) -> fir_col_async7/11(real6)
  fir_col_async6/12(imag_out6) -> fir_col_async7/12(imag6)
  fir_col_async6/13(real_out7) -> fir_col_async7/13(real7)
  fir_col_async6/14(imag_out7) -> fir_col_async7/14(imag7)
  fir_col_async6/15(real_out8) -> fir_col_async7/15(real8)
  fir_col_async6/16(imag_out8) -> fir_col_async7/16(imag8)
  fir_col_async7/33(real_sum) -> real_sum/8(din7)
  fir_col_async7/34(imag_sum) -> imag_sum/8(din7)
  fir_col_async7/1(real_out1) -> fir_col_async8/1(real1)
  fir_col_async7/2(imag_out1) -> fir_col_async8/2(imag1)
  fir_col_async7/3(real_out2) -> fir_col_async8/3(real2)
  fir_col_async7/4(imag_out2) -> fir_col_async8/4(imag2)
  fir_col_async7/5(real_out3) -> fir_col_async8/5(real3)
  fir_col_async7/6(imag_out3) -> fir_col_async8/6(imag3)
  fir_col_async7/7(real_out4) -> fir_col_async8/7(real4)
  fir_col_async7/8(imag_out4) -> fir_col_async8/8(imag4)
  fir_col_async7/9(real_out5) -> fir_col_async8/9(real5)
  fir_col_async7/10(imag_out5) -> fir_col_async8/10(imag5)
  fir_col_async7/11(real_out6) -> fir_col_async8/11(real6)
  fir_col_async7/12(imag_out6) -> fir_col_async8/12(imag6)
  fir_col_async7/13(real_out7) -> fir_col_async8/13(real7)
  fir_col_async7/14(imag_out7) -> fir_col_async8/14(imag7)
  fir_col_async7/15(real_out8) -> fir_col_async8/15(real8)
  fir_col_async7/16(imag_out8) -> fir_col_async8/16(imag8)
  fir_col_async8/33(real_sum) -> real_sum/9(din8)
  fir_col_async8/34(imag_sum) -> imag_sum/9(din8)
  fir_col_async8/1(real_out1) -> fir_col_async9/1(real1)
  fir_col_async8/2(imag_out1) -> fir_col_async9/2(imag1)
  fir_col_async8/3(real_out2) -> fir_col_async9/3(real2)
  fir_col_async8/4(imag_out2) -> fir_col_async9/4(imag2)
  fir_col_async8/5(real_out3) -> fir_col_async9/5(real3)
  fir_col_async8/6(imag_out3) -> fir_col_async9/6(imag3)
  fir_col_async8/7(real_out4) -> fir_col_async9/7(real4)
  fir_col_async8/8(imag_out4) -> fir_col_async9/8(imag4)
  fir_col_async8/9(real_out5) -> fir_col_async9/9(real5)
  fir_col_async8/10(imag_out5) -> fir_col_async9/10(imag5)
  fir_col_async8/11(real_out6) -> fir_col_async9/11(real6)
  fir_col_async8/12(imag_out6) -> fir_col_async9/12(imag6)
  fir_col_async8/13(real_out7) -> fir_col_async9/13(real7)
  fir_col_async8/14(imag_out7) -> fir_col_async9/14(imag7)
  fir_col_async8/15(real_out8) -> fir_col_async9/15(real8)
  fir_col_async8/16(imag_out8) -> fir_col_async9/16(imag8)
  fir_col_async9/33(real_sum) -> real_sum/10(din9)
  fir_col_async9/34(imag_sum) -> imag_sum/10(din9)
  fir_col_async9/1(real_out1) -> fir_col_async10/1(real1)
  fir_col_async9/2(imag_out1) -> fir_col_async10/2(imag1)
  fir_col_async9/3(real_out2) -> fir_col_async10/3(real2)
  fir_col_async9/4(imag_out2) -> fir_col_async10/4(imag2)
  fir_col_async9/5(real_out3) -> fir_col_async10/5(real3)
  fir_col_async9/6(imag_out3) -> fir_col_async10/6(imag3)
  fir_col_async9/7(real_out4) -> fir_col_async10/7(real4)
  fir_col_async9/8(imag_out4) -> fir_col_async10/8(imag4)
  fir_col_async9/9(real_out5) -> fir_col_async10/9(real5)
  fir_col_async9/10(imag_out5) -> fir_col_async10/10(imag5)
  fir_col_async9/11(real_out6) -> fir_col_async10/11(real6)
  fir_col_async9/12(imag_out6) -> fir_col_async10/12(imag6)
  fir_col_async9/13(real_out7) -> fir_col_async10/13(real7)
  fir_col_async9/14(imag_out7) -> fir_col_async10/14(imag7)
  fir_col_async9/15(real_out8) -> fir_col_async10/15(real8)
  fir_col_async9/16(imag_out8) -> fir_col_async10/16(imag8)
  fir_col_async10/33(real_sum) -> real_sum/11(din10)
  fir_col_async10/34(imag_sum) -> imag_sum/11(din10)
  fir_col_async10/1(real_out1) -> fir_col_async11/1(real1)
  fir_col_async10/2(imag_out1) -> fir_col_async11/2(imag1)
  fir_col_async10/3(real_out2) -> fir_col_async11/3(real2)
  fir_col_async10/4(imag_out2) -> fir_col_async11/4(imag2)
  fir_col_async10/5(real_out3) -> fir_col_async11/5(real3)
  fir_col_async10/6(imag_out3) -> fir_col_async11/6(imag3)
  fir_col_async10/7(real_out4) -> fir_col_async11/7(real4)
  fir_col_async10/8(imag_out4) -> fir_col_async11/8(imag4)
  fir_col_async10/9(real_out5) -> fir_col_async11/9(real5)
  fir_col_async10/10(imag_out5) -> fir_col_async11/10(imag5)
  fir_col_async10/11(real_out6) -> fir_col_async11/11(real6)
  fir_col_async10/12(imag_out6) -> fir_col_async11/12(imag6)
  fir_col_async10/13(real_out7) -> fir_col_async11/13(real7)
  fir_col_async10/14(imag_out7) -> fir_col_async11/14(imag7)
  fir_col_async10/15(real_out8) -> fir_col_async11/15(real8)
  fir_col_async10/16(imag_out8) -> fir_col_async11/16(imag8)
  fir_col_async11/33(real_sum) -> real_sum/12(din11)
  fir_col_async11/34(imag_sum) -> imag_sum/12(din11)
  fir_col_async11/1(real_out1) -> fir_col_async12/1(real1)
  fir_col_async11/2(imag_out1) -> fir_col_async12/2(imag1)
  fir_col_async11/3(real_out2) -> fir_col_async12/3(real2)
  fir_col_async11/4(imag_out2) -> fir_col_async12/4(imag2)
  fir_col_async11/5(real_out3) -> fir_col_async12/5(real3)
  fir_col_async11/6(imag_out3) -> fir_col_async12/6(imag3)
  fir_col_async11/7(real_out4) -> fir_col_async12/7(real4)
  fir_col_async11/8(imag_out4) -> fir_col_async12/8(imag4)
  fir_col_async11/9(real_out5) -> fir_col_async12/9(real5)
  fir_col_async11/10(imag_out5) -> fir_col_async12/10(imag5)
  fir_col_async11/11(real_out6) -> fir_col_async12/11(real6)
  fir_col_async11/12(imag_out6) -> fir_col_async12/12(imag6)
  fir_col_async11/13(real_out7) -> fir_col_async12/13(real7)
  fir_col_async11/14(imag_out7) -> fir_col_async12/14(imag7)
  fir_col_async11/15(real_out8) -> fir_col_async12/15(real8)
  fir_col_async11/16(imag_out8) -> fir_col_async12/16(imag8)
  fir_col_async12/33(real_sum) -> real_sum/13(din12)
  fir_col_async12/34(imag_sum) -> imag_sum/13(din12)
  fir_col_async12/1(real_out1) -> fir_col_async13/1(real1)
  fir_col_async12/2(imag_out1) -> fir_col_async13/2(imag1)
  fir_col_async12/3(real_out2) -> fir_col_async13/3(real2)
  fir_col_async12/4(imag_out2) -> fir_col_async13/4(imag2)
  fir_col_async12/5(real_out3) -> fir_col_async13/5(real3)
  fir_col_async12/6(imag_out3) -> fir_col_async13/6(imag3)
  fir_col_async12/7(real_out4) -> fir_col_async13/7(real4)
  fir_col_async12/8(imag_out4) -> fir_col_async13/8(imag4)
  fir_col_async12/9(real_out5) -> fir_col_async13/9(real5)
  fir_col_async12/10(imag_out5) -> fir_col_async13/10(imag5)
  fir_col_async12/11(real_out6) -> fir_col_async13/11(real6)
  fir_col_async12/12(imag_out6) -> fir_col_async13/12(imag6)
  fir_col_async12/13(real_out7) -> fir_col_async13/13(real7)
  fir_col_async12/14(imag_out7) -> fir_col_async13/14(imag7)
  fir_col_async12/15(real_out8) -> fir_col_async13/15(real8)
  fir_col_async12/16(imag_out8) -> fir_col_async13/16(imag8)
  fir_col_async13/33(real_sum) -> real_sum/14(din13)
  fir_col_async13/34(imag_sum) -> imag_sum/14(din13)
  fir_col_async13/1(real_out1) -> fir_col_async14/1(real1)
  fir_col_async13/2(imag_out1) -> fir_col_async14/2(imag1)
  fir_col_async13/3(real_out2) -> fir_col_async14/3(real2)
  fir_col_async13/4(imag_out2) -> fir_col_async14/4(imag2)
  fir_col_async13/5(real_out3) -> fir_col_async14/5(real3)
  fir_col_async13/6(imag_out3) -> fir_col_async14/6(imag3)
  fir_col_async13/7(real_out4) -> fir_col_async14/7(real4)
  fir_col_async13/8(imag_out4) -> fir_col_async14/8(imag4)
  fir_col_async13/9(real_out5) -> fir_col_async14/9(real5)
  fir_col_async13/10(imag_out5) -> fir_col_async14/10(imag5)
  fir_col_async13/11(real_out6) -> fir_col_async14/11(real6)
  fir_col_async13/12(imag_out6) -> fir_col_async14/12(imag6)
  fir_col_async13/13(real_out7) -> fir_col_async14/13(real7)
  fir_col_async13/14(imag_out7) -> fir_col_async14/14(imag7)
  fir_col_async13/15(real_out8) -> fir_col_async14/15(real8)
  fir_col_async13/16(imag_out8) -> fir_col_async14/16(imag8)
  fir_col_async14/33(real_sum) -> real_sum/15(din14)
  fir_col_async14/34(imag_sum) -> imag_sum/15(din14)
  fir_col_async14/1(real_out1) -> fir_col_async15/1(real1)
  fir_col_async14/2(imag_out1) -> fir_col_async15/2(imag1)
  fir_col_async14/3(real_out2) -> fir_col_async15/3(real2)
  fir_col_async14/4(imag_out2) -> fir_col_async15/4(imag2)
  fir_col_async14/5(real_out3) -> fir_col_async15/5(real3)
  fir_col_async14/6(imag_out3) -> fir_col_async15/6(imag3)
  fir_col_async14/7(real_out4) -> fir_col_async15/7(real4)
  fir_col_async14/8(imag_out4) -> fir_col_async15/8(imag4)
  fir_col_async14/9(real_out5) -> fir_col_async15/9(real5)
  fir_col_async14/10(imag_out5) -> fir_col_async15/10(imag5)
  fir_col_async14/11(real_out6) -> fir_col_async15/11(real6)
  fir_col_async14/12(imag_out6) -> fir_col_async15/12(imag6)
  fir_col_async14/13(real_out7) -> fir_col_async15/13(real7)
  fir_col_async14/14(imag_out7) -> fir_col_async15/14(imag7)
  fir_col_async14/15(real_out8) -> fir_col_async15/15(real8)
  fir_col_async14/16(imag_out8) -> fir_col_async15/16(imag8)
  fir_col_async15/33(real_sum) -> real_sum/16(din15)
  fir_col_async15/34(imag_sum) -> imag_sum/16(din15)
  fir_col_async15/1(real_out1) -> fir_col_async16/1(real1)
  fir_col_async15/2(imag_out1) -> fir_col_async16/2(imag1)
  fir_col_async15/3(real_out2) -> fir_col_async16/3(real2)
  fir_col_async15/4(imag_out2) -> fir_col_async16/4(imag2)
  fir_col_async15/5(real_out3) -> fir_col_async16/5(real3)
  fir_col_async15/6(imag_out3) -> fir_col_async16/6(imag3)
  fir_col_async15/7(real_out4) -> fir_col_async16/7(real4)
  fir_col_async15/8(imag_out4) -> fir_col_async16/8(imag4)
  fir_col_async15/9(real_out5) -> fir_col_async16/9(real5)
  fir_col_async15/10(imag_out5) -> fir_col_async16/10(imag5)
  fir_col_async15/11(real_out6) -> fir_col_async16/11(real6)
  fir_col_async15/12(imag_out6) -> fir_col_async16/12(imag6)
  fir_col_async15/13(real_out7) -> fir_col_async16/13(real7)
  fir_col_async15/14(imag_out7) -> fir_col_async16/14(imag7)
  fir_col_async15/15(real_out8) -> fir_col_async16/15(real8)
  fir_col_async15/16(imag_out8) -> fir_col_async16/16(imag8)
  fir_col_async16/33(real_sum) -> real_sum/17(din16)
  fir_col_async16/34(imag_sum) -> imag_sum/17(din16)
  real_sum/2(dout) -> shift1/1
  imag_sum/2(dout) -> shift2/1
  shift1/1 -> convert1/1
  shift2/1 -> convert2/1
  convert1/1 -> ri_to_c/1
  convert2/1 -> ri_to_c/2
  ri_to_c/1 -> dout/1
  sync_delay/1 -> real_sum/1(sync), imag_sum/1(sync)
  real_sum/1(sync_out) -> sync_out/1
  fir_col_async2/17(real_back_out1) -> fir_col_async1/17(real_back1)
  fir_col_async2/18(imag_back_out1) -> fir_col_async1/18(imag_back1)
  fir_col_async2/19(real_back_out2) -> fir_col_async1/19(real_back2)
  fir_col_async2/20(imag_back_out2) -> fir_col_async1/20(imag_back2)
  fir_col_async2/21(real_back_out3) -> fir_col_async1/21(real_back3)
  fir_col_async2/22(imag_back_out3) -> fir_col_async1/22(imag_back3)
  fir_col_async2/23(real_back_out4) -> fir_col_async1/23(real_back4)
  fir_col_async2/24(imag_back_out4) -> fir_col_async1/24(imag_back4)
  fir_col_async2/25(real_back_out5) -> fir_col_async1/25(real_back5)
  fir_col_async2/26(imag_back_out5) -> fir_col_async1/26(imag_back5)
  fir_col_async2/27(real_back_out6) -> fir_col_async1/27(real_back6)
  fir_col_async2/28(imag_back_out6) -> fir_col_async1/28(imag_back6)
  fir_col_async2/29(real_back_out7) -> fir_col_async1/29(real_back7)
  fir_col_async2/30(imag_back_out7) -> fir_col_async1/30(imag_back7)
  fir_col_async2/31(real_back_out8) -> fir_col_async1/31(real_back8)
  fir_col_async2/32(imag_back_out8) -> fir_col_async1/32(imag_back8)
  fir_col_async3/17(real_back_out1) -> fir_col_async2/17(real_back1)
  fir_col_async3/18(imag_back_out1) -> fir_col_async2/18(imag_back1)
  fir_col_async3/19(real_back_out2) -> fir_col_async2/19(real_back2)
  fir_col_async3/20(imag_back_out2) -> fir_col_async2/20(imag_back2)
  fir_col_async3/21(real_back_out3) -> fir_col_async2/21(real_back3)
  fir_col_async3/22(imag_back_out3) -> fir_col_async2/22(imag_back3)
  fir_col_async3/23(real_back_out4) -> fir_col_async2/23(real_back4)
  fir_col_async3/24(imag_back_out4) -> fir_col_async2/24(imag_back4)
  fir_col_async3/25(real_back_out5) -> fir_col_async2/25(real_back5)
  fir_col_async3/26(imag_back_out5) -> fir_col_async2/26(imag_back5)
  fir_col_async3/27(real_back_out6) -> fir_col_async2/27(real_back6)
  fir_col_async3/28(imag_back_out6) -> fir_col_async2/28(imag_back6)
  fir_col_async3/29(real_back_out7) -> fir_col_async2/29(real_back7)
  fir_col_async3/30(imag_back_out7) -> fir_col_async2/30(imag_back7)
  fir_col_async3/31(real_back_out8) -> fir_col_async2/31(real_back8)
  fir_col_async3/32(imag_back_out8) -> fir_col_async2/32(imag_back8)
  fir_col_async4/17(real_back_out1) -> fir_col_async3/17(real_back1)
  fir_col_async4/18(imag_back_out1) -> fir_col_async3/18(imag_back1)
  fir_col_async4/19(real_back_out2) -> fir_col_async3/19(real_back2)
  fir_col_async4/20(imag_back_out2) -> fir_col_async3/20(imag_back2)
  fir_col_async4/21(real_back_out3) -> fir_col_async3/21(real_back3)
  fir_col_async4/22(imag_back_out3) -> fir_col_async3/22(imag_back3)
  fir_col_async4/23(real_back_out4) -> fir_col_async3/23(real_back4)
  fir_col_async4/24(imag_back_out4) -> fir_col_async3/24(imag_back4)
  fir_col_async4/25(real_back_out5) -> fir_col_async3/25(real_back5)
  fir_col_async4/26(imag_back_out5) -> fir_col_async3/26(imag_back5)
  fir_col_async4/27(real_back_out6) -> fir_col_async3/27(real_back6)
  fir_col_async4/28(imag_back_out6) -> fir_col_async3/28(imag_back6)
  fir_col_async4/29(real_back_out7) -> fir_col_async3/29(real_back7)
  fir_col_async4/30(imag_back_out7) -> fir_col_async3/30(imag_back7)
  fir_col_async4/31(real_back_out8) -> fir_col_async3/31(real_back8)
  fir_col_async4/32(imag_back_out8) -> fir_col_async3/32(imag_back8)
  fir_col_async5/17(real_back_out1) -> fir_col_async4/17(real_back1)
  fir_col_async5/18(imag_back_out1) -> fir_col_async4/18(imag_back1)
  fir_col_async5/19(real_back_out2) -> fir_col_async4/19(real_back2)
  fir_col_async5/20(imag_back_out2) -> fir_col_async4/20(imag_back2)
  fir_col_async5/21(real_back_out3) -> fir_col_async4/21(real_back3)
  fir_col_async5/22(imag_back_out3) -> fir_col_async4/22(imag_back3)
  fir_col_async5/23(real_back_out4) -> fir_col_async4/23(real_back4)
  fir_col_async5/24(imag_back_out4) -> fir_col_async4/24(imag_back4)
  fir_col_async5/25(real_back_out5) -> fir_col_async4/25(real_back5)
  fir_col_async5/26(imag_back_out5) -> fir_col_async4/26(imag_back5)
  fir_col_async5/27(real_back_out6) -> fir_col_async4/27(real_back6)
  fir_col_async5/28(imag_back_out6) -> fir_col_async4/28(imag_back6)
  fir_col_async5/29(real_back_out7) -> fir_col_async4/29(real_back7)
  fir_col_async5/30(imag_back_out7) -> fir_col_async4/30(imag_back7)
  fir_col_async5/31(real_back_out8) -> fir_col_async4/31(real_back8)
  fir_col_async5/32(imag_back_out8) -> fir_col_async4/32(imag_back8)
  fir_col_async6/17(real_back_out1) -> fir_col_async5/17(real_back1)
  fir_col_async6/18(imag_back_out1) -> fir_col_async5/18(imag_back1)
  fir_col_async6/19(real_back_out2) -> fir_col_async5/19(real_back2)
  fir_col_async6/20(imag_back_out2) -> fir_col_async5/20(imag_back2)
  fir_col_async6/21(real_back_out3) -> fir_col_async5/21(real_back3)
  fir_col_async6/22(imag_back_out3) -> fir_col_async5/22(imag_back3)
  fir_col_async6/23(real_back_out4) -> fir_col_async5/23(real_back4)
  fir_col_async6/24(imag_back_out4) -> fir_col_async5/24(imag_back4)
  fir_col_async6/25(real_back_out5) -> fir_col_async5/25(real_back5)
  fir_col_async6/26(imag_back_out5) -> fir_col_async5/26(imag_back5)
  fir_col_async6/27(real_back_out6) -> fir_col_async5/27(real_back6)
  fir_col_async6/28(imag_back_out6) -> fir_col_async5/28(imag_back6)
  fir_col_async6/29(real_back_out7) -> fir_col_async5/29(real_back7)
  fir_col_async6/30(imag_back_out7) -> fir_col_async5/30(imag_back7)
  fir_col_async6/31(real_back_out8) -> fir_col_async5/31(real_back8)
  fir_col_async6/32(imag_back_out8) -> fir_col_async5/32(imag_back8)
  fir_col_async7/17(real_back_out1) -> fir_col_async6/17(real_back1)
  fir_col_async7/18(imag_back_out1) -> fir_col_async6/18(imag_back1)
  fir_col_async7/19(real_back_out2) -> fir_col_async6/19(real_back2)
  fir_col_async7/20(imag_back_out2) -> fir_col_async6/20(imag_back2)
  fir_col_async7/21(real_back_out3) -> fir_col_async6/21(real_back3)
  fir_col_async7/22(imag_back_out3) -> fir_col_async6/22(imag_back3)
  fir_col_async7/23(real_back_out4) -> fir_col_async6/23(real_back4)
  fir_col_async7/24(imag_back_out4) -> fir_col_async6/24(imag_back4)
  fir_col_async7/25(real_back_out5) -> fir_col_async6/25(real_back5)
  fir_col_async7/26(imag_back_out5) -> fir_col_async6/26(imag_back5)
  fir_col_async7/27(real_back_out6) -> fir_col_async6/27(real_back6)
  fir_col_async7/28(imag_back_out6) -> fir_col_async6/28(imag_back6)
  fir_col_async7/29(real_back_out7) -> fir_col_async6/29(real_back7)
  fir_col_async7/30(imag_back_out7) -> fir_col_async6/30(imag_back7)
  fir_col_async7/31(real_back_out8) -> fir_col_async6/31(real_back8)
  fir_col_async7/32(imag_back_out8) -> fir_col_async6/32(imag_back8)
  fir_col_async8/17(real_back_out1) -> fir_col_async7/17(real_back1)
  fir_col_async8/18(imag_back_out1) -> fir_col_async7/18(imag_back1)
  fir_col_async8/19(real_back_out2) -> fir_col_async7/19(real_back2)
  fir_col_async8/20(imag_back_out2) -> fir_col_async7/20(imag_back2)
  fir_col_async8/21(real_back_out3) -> fir_col_async7/21(real_back3)
  fir_col_async8/22(imag_back_out3) -> fir_col_async7/22(imag_back3)
  fir_col_async8/23(real_back_out4) -> fir_col_async7/23(real_back4)
  fir_col_async8/24(imag_back_out4) -> fir_col_async7/24(imag_back4)
  fir_col_async8/25(real_back_out5) -> fir_col_async7/25(real_back5)
  fir_col_async8/26(imag_back_out5) -> fir_col_async7/26(imag_back5)
  fir_col_async8/27(real_back_out6) -> fir_col_async7/27(real_back6)
  fir_col_async8/28(imag_back_out6) -> fir_col_async7/28(imag_back6)
  fir_col_async8/29(real_back_out7) -> fir_col_async7/29(real_back7)
  fir_col_async8/30(imag_back_out7) -> fir_col_async7/30(imag_back7)
  fir_col_async8/31(real_back_out8) -> fir_col_async7/31(real_back8)
  fir_col_async8/32(imag_back_out8) -> fir_col_async7/32(imag_back8)
  fir_col_async9/17(real_back_out1) -> fir_col_async8/17(real_back1)
  fir_col_async9/18(imag_back_out1) -> fir_col_async8/18(imag_back1)
  fir_col_async9/19(real_back_out2) -> fir_col_async8/19(real_back2)
  fir_col_async9/20(imag_back_out2) -> fir_col_async8/20(imag_back2)
  fir_col_async9/21(real_back_out3) -> fir_col_async8/21(real_back3)
  fir_col_async9/22(imag_back_out3) -> fir_col_async8/22(imag_back3)
  fir_col_async9/23(real_back_out4) -> fir_col_async8/23(real_back4)
  fir_col_async9/24(imag_back_out4) -> fir_col_async8/24(imag_back4)
  fir_col_async9/25(real_back_out5) -> fir_col_async8/25(real_back5)
  fir_col_async9/26(imag_back_out5) -> fir_col_async8/26(imag_back5)
  fir_col_async9/27(real_back_out6) -> fir_col_async8/27(real_back6)
  fir_col_async9/28(imag_back_out6) -> fir_col_async8/28(imag_back6)
  fir_col_async9/29(real_back_out7) -> fir_col_async8/29(real_back7)
  fir_col_async9/30(imag_back_out7) -> fir_col_async8/30(imag_back7)
  fir_col_async9/31(real_back_out8) -> fir_col_async8/31(real_back8)
  fir_col_async9/32(imag_back_out8) -> fir_col_async8/32(imag_back8)
  fir_col_async10/17(real_back_out1) -> fir_col_async9/17(real_back1)
  fir_col_async10/18(imag_back_out1) -> fir_col_async9/18(imag_back1)
  fir_col_async10/19(real_back_out2) -> fir_col_async9/19(real_back2)
  fir_col_async10/20(imag_back_out2) -> fir_col_async9/20(imag_back2)
  fir_col_async10/21(real_back_out3) -> fir_col_async9/21(real_back3)
  fir_col_async10/22(imag_back_out3) -> fir_col_async9/22(imag_back3)
  fir_col_async10/23(real_back_out4) -> fir_col_async9/23(real_back4)
  fir_col_async10/24(imag_back_out4) -> fir_col_async9/24(imag_back4)
  fir_col_async10/25(real_back_out5) -> fir_col_async9/25(real_back5)
  fir_col_async10/26(imag_back_out5) -> fir_col_async9/26(imag_back5)
  fir_col_async10/27(real_back_out6) -> fir_col_async9/27(real_back6)
  fir_col_async10/28(imag_back_out6) -> fir_col_async9/28(imag_back6)
  fir_col_async10/29(real_back_out7) -> fir_col_async9/29(real_back7)
  fir_col_async10/30(imag_back_out7) -> fir_col_async9/30(imag_back7)
  fir_col_async10/31(real_back_out8) -> fir_col_async9/31(real_back8)
  fir_col_async10/32(imag_back_out8) -> fir_col_async9/32(imag_back8)
  fir_col_async11/17(real_back_out1) -> fir_col_async10/17(real_back1)
  fir_col_async11/18(imag_back_out1) -> fir_col_async10/18(imag_back1)
  fir_col_async11/19(real_back_out2) -> fir_col_async10/19(real_back2)
  fir_col_async11/20(imag_back_out2) -> fir_col_async10/20(imag_back2)
  fir_col_async11/21(real_back_out3) -> fir_col_async10/21(real_back3)
  fir_col_async11/22(imag_back_out3) -> fir_col_async10/22(imag_back3)
  fir_col_async11/23(real_back_out4) -> fir_col_async10/23(real_back4)
  fir_col_async11/24(imag_back_out4) -> fir_col_async10/24(imag_back4)
  fir_col_async11/25(real_back_out5) -> fir_col_async10/25(real_back5)
  fir_col_async11/26(imag_back_out5) -> fir_col_async10/26(imag_back5)
  fir_col_async11/27(real_back_out6) -> fir_col_async10/27(real_back6)
  fir_col_async11/28(imag_back_out6) -> fir_col_async10/28(imag_back6)
  fir_col_async11/29(real_back_out7) -> fir_col_async10/29(real_back7)
  fir_col_async11/30(imag_back_out7) -> fir_col_async10/30(imag_back7)
  fir_col_async11/31(real_back_out8) -> fir_col_async10/31(real_back8)
  fir_col_async11/32(imag_back_out8) -> fir_col_async10/32(imag_back8)
  fir_col_async12/17(real_back_out1) -> fir_col_async11/17(real_back1)
  fir_col_async12/18(imag_back_out1) -> fir_col_async11/18(imag_back1)
  fir_col_async12/19(real_back_out2) -> fir_col_async11/19(real_back2)
  fir_col_async12/20(imag_back_out2) -> fir_col_async11/20(imag_back2)
  fir_col_async12/21(real_back_out3) -> fir_col_async11/21(real_back3)
  fir_col_async12/22(imag_back_out3) -> fir_col_async11/22(imag_back3)
  fir_col_async12/23(real_back_out4) -> fir_col_async11/23(real_back4)
  fir_col_async12/24(imag_back_out4) -> fir_col_async11/24(imag_back4)
  fir_col_async12/25(real_back_out5) -> fir_col_async11/25(real_back5)
  fir_col_async12/26(imag_back_out5) -> fir_col_async11/26(imag_back5)
  fir_col_async12/27(real_back_out6) -> fir_col_async11/27(real_back6)
  fir_col_async12/28(imag_back_out6) -> fir_col_async11/28(imag_back6)
  fir_col_async12/29(real_back_out7) -> fir_col_async11/29(real_back7)
  fir_col_async12/30(imag_back_out7) -> fir_col_async11/30(imag_back7)
  fir_col_async12/31(real_back_out8) -> fir_col_async11/31(real_back8)
  fir_col_async12/32(imag_back_out8) -> fir_col_async11/32(imag_back8)
  fir_col_async13/17(real_back_out1) -> fir_col_async12/17(real_back1)
  fir_col_async13/18(imag_back_out1) -> fir_col_async12/18(imag_back1)
  fir_col_async13/19(real_back_out2) -> fir_col_async12/19(real_back2)
  fir_col_async13/20(imag_back_out2) -> fir_col_async12/20(imag_back2)
  fir_col_async13/21(real_back_out3) -> fir_col_async12/21(real_back3)
  fir_col_async13/22(imag_back_out3) -> fir_col_async12/22(imag_back3)
  fir_col_async13/23(real_back_out4) -> fir_col_async12/23(real_back4)
  fir_col_async13/24(imag_back_out4) -> fir_col_async12/24(imag_back4)
  fir_col_async13/25(real_back_out5) -> fir_col_async12/25(real_back5)
  fir_col_async13/26(imag_back_out5) -> fir_col_async12/26(imag_back5)
  fir_col_async13/27(real_back_out6) -> fir_col_async12/27(real_back6)
  fir_col_async13/28(imag_back_out6) -> fir_col_async12/28(imag_back6)
  fir_col_async13/29(real_back_out7) -> fir_col_async12/29(real_back7)
  fir_col_async13/30(imag_back_out7) -> fir_col_async12/30(imag_back7)
  fir_col_async13/31(real_back_out8) -> fir_col_async12/31(real_back8)
  fir_col_async13/32(imag_back_out8) -> fir_col_async12/32(imag_back8)
  fir_col_async14/17(real_back_out1) -> fir_col_async13/17(real_back1)
  fir_col_async14/18(imag_back_out1) -> fir_col_async13/18(imag_back1)
  fir_col_async14/19(real_back_out2) -> fir_col_async13/19(real_back2)
  fir_col_async14/20(imag_back_out2) -> fir_col_async13/20(imag_back2)
  fir_col_async14/21(real_back_out3) -> fir_col_async13/21(real_back3)
  fir_col_async14/22(imag_back_out3) -> fir_col_async13/22(imag_back3)
  fir_col_async14/23(real_back_out4) -> fir_col_async13/23(real_back4)
  fir_col_async14/24(imag_back_out4) -> fir_col_async13/24(imag_back4)
  fir_col_async14/25(real_back_out5) -> fir_col_async13/25(real_back5)
  fir_col_async14/26(imag_back_out5) -> fir_col_async13/26(imag_back5)
  fir_col_async14/27(real_back_out6) -> fir_col_async13/27(real_back6)
  fir_col_async14/28(imag_back_out6) -> fir_col_async13/28(imag_back6)
  fir_col_async14/29(real_back_out7) -> fir_col_async13/29(real_back7)
  fir_col_async14/30(imag_back_out7) -> fir_col_async13/30(imag_back7)
  fir_col_async14/31(real_back_out8) -> fir_col_async13/31(real_back8)
  fir_col_async14/32(imag_back_out8) -> fir_col_async13/32(imag_back8)
  fir_col_async15/17(real_back_out1) -> fir_col_async14/17(real_back1)
  fir_col_async15/18(imag_back_out1) -> fir_col_async14/18(imag_back1)
  fir_col_async15/19(real_back_out2) -> fir_col_async14/19(real_back2)
  fir_col_async15/20(imag_back_out2) -> fir_col_async14/20(imag_back2)
  fir_col_async15/21(real_back_out3) -> fir_col_async14/21(real_back3)
  fir_col_async15/22(imag_back_out3) -> fir_col_async14/22(imag_back3)
  fir_col_async15/23(real_back_out4) -> fir_col_async14/23(real_back4)
  fir_col_async15/24(imag_back_out4) -> fir_col_async14/24(imag_back4)
  fir_col_async15/25(real_back_out5) -> fir_col_async14/25(real_back5)
  fir_col_async15/26(imag_back_out5) -> fir_col_async14/26(imag_back5)
  fir_col_async15/27(real_back_out6) -> fir_col_async14/27(real_back6)
  fir_col_async15/28(imag_back_out6) -> fir_col_async14/28(imag_back6)
  fir_col_async15/29(real_back_out7) -> fir_col_async14/29(real_back7)
  fir_col_async15/30(imag_back_out7) -> fir_col_async14/30(imag_back7)
  fir_col_async15/31(real_back_out8) -> fir_col_async14/31(real_back8)
  fir_col_async15/32(imag_back_out8) -> fir_col_async14/32(imag_back8)
  fir_col_async16/17(real_back_out1) -> fir_col_async15/17(real_back1)
  fir_col_async16/18(imag_back_out1) -> fir_col_async15/18(imag_back1)
  fir_col_async16/19(real_back_out2) -> fir_col_async15/19(real_back2)
  fir_col_async16/20(imag_back_out2) -> fir_col_async15/20(imag_back2)
  fir_col_async16/21(real_back_out3) -> fir_col_async15/21(real_back3)
  fir_col_async16/22(imag_back_out3) -> fir_col_async15/22(imag_back3)
  fir_col_async16/23(real_back_out4) -> fir_col_async15/23(real_back4)
  fir_col_async16/24(imag_back_out4) -> fir_col_async15/24(imag_back4)
  fir_col_async16/25(real_back_out5) -> fir_col_async15/25(real_back5)
  fir_col_async16/26(imag_back_out5) -> fir_col_async15/26(imag_back5)
  fir_col_async16/27(real_back_out6) -> fir_col_async15/27(real_back6)
  fir_col_async16/28(imag_back_out6) -> fir_col_async15/28(imag_back6)
  fir_col_async16/29(real_back_out7) -> fir_col_async15/29(real_back7)
  fir_col_async16/30(imag_back_out7) -> fir_col_async15/30(imag_back7)
  fir_col_async16/31(real_back_out8) -> fir_col_async15/31(real_back8)
  fir_col_async16/32(imag_back_out8) -> fir_col_async15/32(imag_back8)
  fir_col_async16/1(real_out1) -> fir_col_async16/17(real_back1)
  fir_col_async16/2(imag_out1) -> fir_col_async16/18(imag_back1)
  fir_col_async16/3(real_out2) -> fir_col_async16/19(real_back2)
  fir_col_async16/4(imag_out2) -> fir_col_async16/20(imag_back2)
  fir_col_async16/5(real_out3) -> fir_col_async16/21(real_back3)
  fir_col_async16/6(imag_out3) -> fir_col_async16/22(imag_back3)
  fir_col_async16/7(real_out4) -> fir_col_async16/23(real_back4)
  fir_col_async16/8(imag_out4) -> fir_col_async16/24(imag_back4)
  fir_col_async16/9(real_out5) -> fir_col_async16/25(real_back5)
  fir_col_async16/10(imag_out5) -> fir_col_async16/26(imag_back5)
  fir_col_async16/11(real_out6) -> fir_col_async16/27(real_back6)
  fir_col_async16/12(imag_out6) -> fir_col_async16/28(imag_back6)
  fir_col_async16/13(real_out7) -> fir_col_async16/29(real_back7)
  fir_col_async16/14(imag_out7) -> fir_col_async16/30(imag_back7)
  fir_col_async16/15(real_out8) -> fir_col_async16/31(real_back8)
  fir_col_async16/16(imag_out8) -> fir_col_async16/32(imag_back8)
